simulink model "model"  (R2025b)
settings: Solver=VariableStepAuto  StartTime=0.0  StopTime=10.0  RelTol=1e-3
settings Model: Creator=maxus  LastModifiedBy=maxus

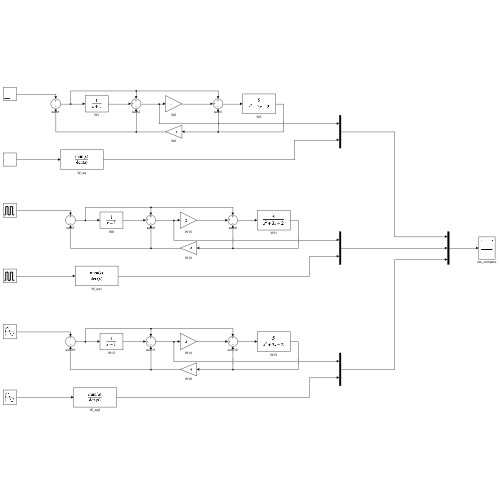
[thumbnail: Simulink's stored preview of the top-level diagram]
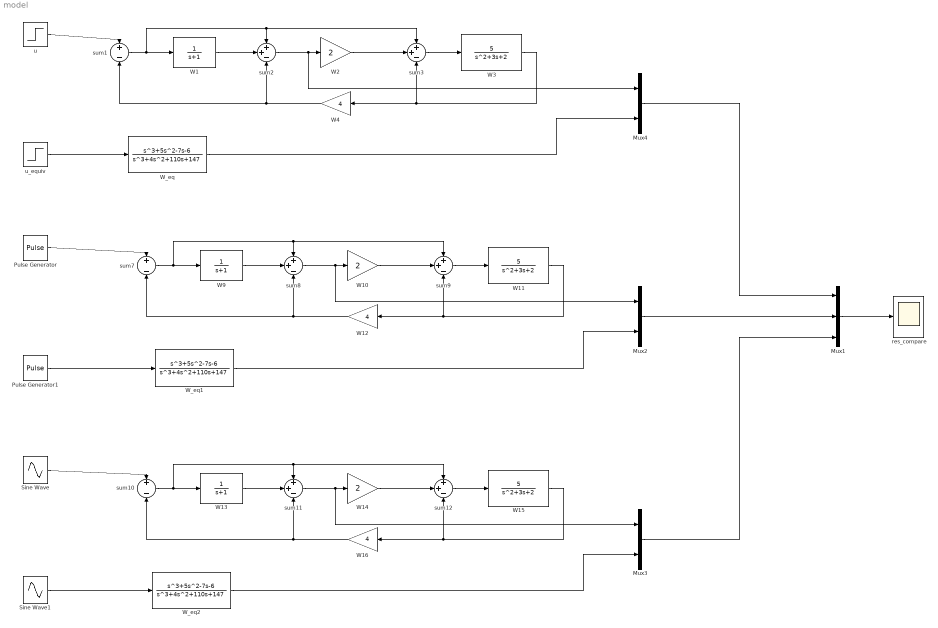
== system model ==
  Mux1 : Mux  Inputs=3
  Mux2 : Mux  Inputs=2
  Mux3 : Mux  Inputs=2
  Mux4 : Mux  Inputs=2
  Pulse Generator : DiscretePulseGenerator  Description=fdfds  PulseType=Time based  Period=10  PulseWidth=5
  Pulse Generator1 : DiscretePulseGenerator  PulseType=Time based  Period=10  PulseWidth=5
  Sine Wave : Sin  SampleTime=0
  Sine Wave1 : Sin  SampleTime=0
  W1 : TransferFcn  Denominator=[1 1]
  W10 : Gain  Gain=2
  W11 : TransferFcn  Numerator=[5]  Denominator=[1 3 2]
  W12 : Gain  Gain=4
  W13 : TransferFcn  Denominator=[1 1]
  W14 : Gain  Gain=2
  W15 : TransferFcn  Numerator=[5]  Denominator=[1 3 2]
  W16 : Gain  Gain=4
  W2 : Gain  Gain=2
  W3 : TransferFcn  Numerator=[5]  Denominator=[1 3 2]
  W4 : Gain  Gain=4
  W9 : TransferFcn  Denominator=[1 1]
  W_eq : TransferFcn  Numerator=[1 5 -7 -6]  Denominator=[1 4 110 147]
  W_eq1 : TransferFcn  Numerator=[1 5 -7 -6]  Denominator=[1 4 110 147]
  W_eq2 : TransferFcn  Numerator=[1 5 -7 -6]  Denominator=[1 4 110 147]
  res_compare : Scope
      settings: ActiveDisplayYMinimum=-1.6771764756896725  ActiveDisplayYMaximum=2.7681366651822774
  sum1 : Sum  Inputs=+-
  sum10 : Sum  Inputs=+-
  sum{2..3,8..9,11..12} (6 alike) : Sum  Inputs=++-
  sum7 : Sum  Inputs=+-
  u : Step  SampleTime=0
  u_equiv : Step  SampleTime=0
  wires:
  Pulse Generator1/1 -> W_eq1/1
  W12/1 -> sum7/2, sum8/3
  W_eq1/1 -> Mux2/2
  sum7/1 -> W9/1, sum9/1, sum8/1
  sum8/1 -> W10/1, Mux2/1
  W9/1 -> sum8/2
  sum9/1 -> W11/1
  W11/1 -> W12/1, sum9/3
  W10/1 -> sum9/2
  Pulse Generator/1 -> sum7/1
  Sine Wave/1 -> sum10/1
  W14/1 -> sum12/2
  W15/1 -> sum12/3, W16/1
  sum12/1 -> W15/1
  W13/1 -> sum11/2
  sum11/1 -> Mux3/1, W14/1
  sum10/1 -> sum11/1, sum12/1, W13/1
  W_eq2/1 -> Mux3/2
  W16/1 -> sum11/3, sum10/2
  Sine Wave1/1 -> W_eq2/1
  u/1 -> sum1/1
  W2/1 -> sum3/2
  W3/1 -> sum3/3, W4/1
  sum3/1 -> W3/1
  W1/1 -> sum2/2
  sum2/1 -> Mux4/1, W2/1
  sum1/1 -> sum2/1, sum3/1, W1/1
  W_eq/1 -> Mux4/2
  W4/1 -> sum2/3, sum1/2
  u_equiv/1 -> W_eq/1
  Mux2/1 -> Mux1/2
  Mux3/1 -> Mux1/3
  Mux1/1 -> res_compare/1
  Mux4/1 -> Mux1/1
